simulink model "DC_Virtual_Bus"  (R2025a)
settings: Solver=VariableStepAuto  StartTime=0.0  StopTime=0.8  RelTol=1e-3
libraries: spsIGBTDiodeLib x5, spsSeriesRLCBranchLib x5, spsVoltageMeasurementLib x2, spsDCVoltageSourceLib x1, spsCurrentMeasurementLib x1, simulink x1, sps_lib x1
settings Model: Creator=Mohamed Ibrahim  LastModifiedBy=Mohamed Ibrahim
settings SolverCC: ZeroCrossAlgorithm=Adaptive
settings DebuggingCC: IgnoredZcDiagnostic=none

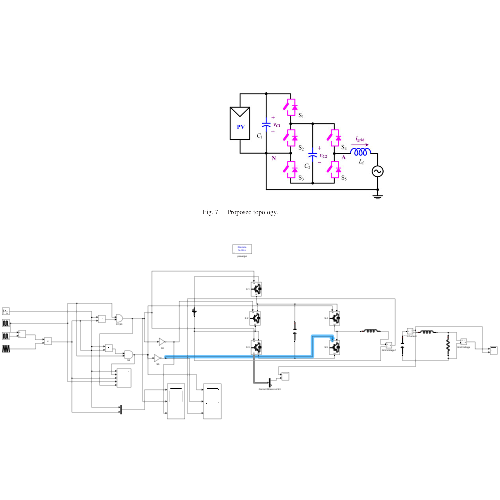
[thumbnail: Simulink's stored preview of the top-level diagram]
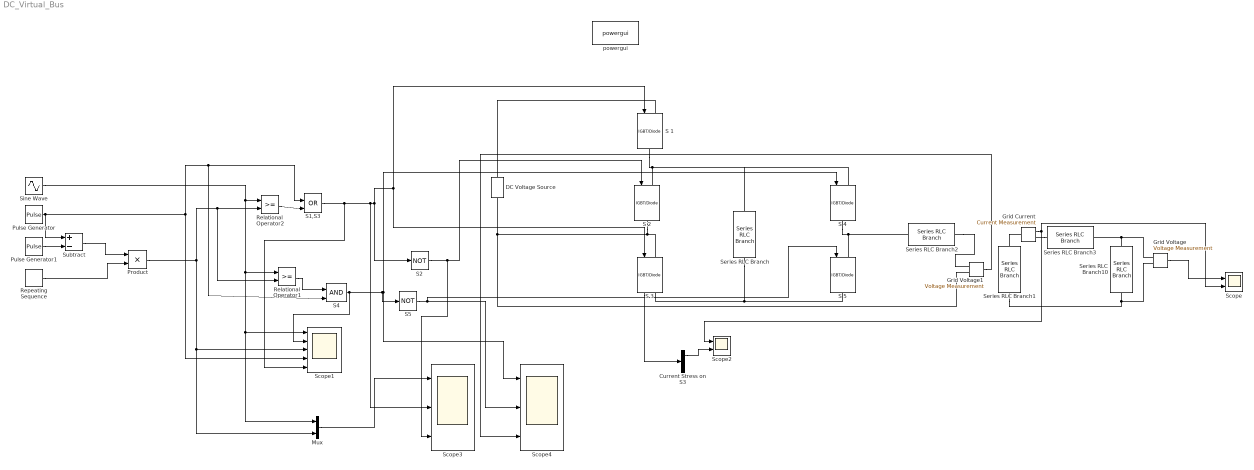
== system DC_Virtual_Bus ==
  Current Stress on S3 : Demux  Outputs=2
  DC Voltage Source : spsDCVoltageSourceLib/DC Voltage Source  Amplitude=400  Measurements=None
  Grid Current : spsCurrentMeasurementLib/Current Measurement  PhasorSimulation=off  OutputType=Complex  PSBequivalent=0
  Grid Voltage : spsVoltageMeasurementLib/Voltage Measurement  PhasorSimulation=off  OutputType=Complex  PSBequivalent=0
  Grid Voltage1 : spsVoltageMeasurementLib/Voltage Measurement  PhasorSimulation=off  OutputType=Complex  PSBequivalent=0
  Mux : Mux  Inputs=2
  Product : Product
  Pulse Generator : DiscretePulseGenerator  PulseType=Time based  Period=0.02  PulseWidth=50
  Pulse Generator1 : DiscretePulseGenerator  PulseType=Time based  Period=0.02  PulseWidth=50  PhaseDelay=0.01
  Relational Operator1 : RelationalOperator  OutDataTypeStr=boolean  RndMeth=Simplest  InputSameDT=off
  Relational Operator2 : RelationalOperator  OutDataTypeStr=boolean  RndMeth=Simplest  InputSameDT=off
  Repeating Sequence : simulink/Sources/Repeating Sequence  rep_seq_t=[0 0.000025 0.00005]  rep_seq_y=[0 1 0]
  S {1..2,4..5} (4 alike) : spsIGBTDiodeLib/IGBT//Diode  Ron=1e-3  Rs=1e5  Cs=inf  Measurements=off
  S 3 : spsIGBTDiodeLib/IGBT//Diode  Ron=1e-3  Rs=1e5  Cs=inf  Measurements=on
  S1,S3 : Logic  Operator=OR  IconShape=distinctive  AllPortsSameDT=off  OutDataTypeStr=boolean
  S2 : Logic  Operator=NOT  IconShape=distinctive  AllPortsSameDT=off  OutDataTypeStr=boolean
  S4 : Logic  IconShape=distinctive  AllPortsSameDT=off  OutDataTypeStr=boolean
  S5 : Logic  Operator=NOT  IconShape=distinctive  AllPortsSameDT=off  OutDataTypeStr=boolean
  Scope : Scope  NumInputPorts=2
      settings: ActiveDisplayYMinimum=-47.58360382260738  ActiveDisplayYMaximum=47.961593181546164
  Scope1 : Scope  NumInputPorts=5
      settings: ActiveDisplayString=4  ActiveDisplayYMinimum=-0.12499999999999997  ActiveDisplayYMaximum=1.125
  Scope2 : Scope  NumInputPorts=2
      settings: ActiveDisplayYMinimum=-47.58360382260738  ActiveDisplayYMaximum=47.961593181546164  DataLoggingVariableName=ScopeData2
  Scope3 : Scope  NumInputPorts=3
      settings: ActiveDisplayYMinimum=-1.25  ActiveDisplayYMaximum=1.25  DataLoggingVariableName=ScopeData3
  Scope4 : Scope  NumInputPorts=3
      settings: ActiveDisplayYMinimum=-0.12499999999999997  ActiveDisplayYMaximum=1.125  DataLoggingVariableName=ScopeData4
  Series RLC Branch : spsSeriesRLCBranchLib/Series RLC Branch  LConnTagsString=__new0  RConnTagsString=__new0  BranchType=C  Resistance=1  Inductance=1e-3  SetiL0=off  InitialCurrent=0  Capacitance=940e-6  Setx0=off  InitialVoltage=0  Measurements=None
  Series RLC Branch1 : spsSeriesRLCBranchLib/Series RLC Branch  LConnTagsString=__new0  RConnTagsString=__new0  BranchType=C  Resistance=1  Inductance=8e-3  SetiL0=off  InitialCurrent=0  Capacitance=0.34e-6  Setx0=off  InitialVoltage=0  Measurements=None
  Series RLC Branch10 : spsSeriesRLCBranchLib/Series RLC Branch  LConnTagsString=__new0  RConnTagsString=__new0  BranchType=R  Resistance=10  Inductance=0.8e-3  SetiL0=off  InitialCurrent=0  Capacitance=1e-6  Setx0=off  InitialVoltage=0  Measurements=None
  Series RLC Branch2 : spsSeriesRLCBranchLib/Series RLC Branch  LConnTagsString=__new0  RConnTagsString=__new0  BranchType=L  Resistance=1  Inductance=8e-3  SetiL0=off  InitialCurrent=0  Capacitance=1e-6  Setx0=off  InitialVoltage=0  Measurements=None
  Series RLC Branch3 : spsSeriesRLCBranchLib/Series RLC Branch  LConnTagsString=__new0  RConnTagsString=__new0  BranchType=L  Resistance=1  Inductance=0.8e-3  SetiL0=off  InitialCurrent=0  Capacitance=1e-6  Setx0=off  InitialVoltage=0  Measurements=None
  Sine Wave : Sin  Frequency=100*pi  SampleTime=0
  Subtract : Sum  Inputs=+-
  powergui : sps_lib/powergui  Priority=1  SimulationMode=Discrete  SampleTime=1e-6  frequency=60  Iterations=50  frequencyindice=0  Pbase=100e6  ErrMax=1e-4  UnitsV=kV  UnitsW=MW  buscounter=0  FunctionMessages=off  echomessages=off  EnableUseOfTLC=off  CurrentSourceSwitches=off  DisableSnubberDevices=off  DisableRonSwitches=off  DisableVfSwitches=off  DisplayEquations=off  AutomaticDiscreteSolvers=off  SolverType=Tustin/Backward Euler (TBE)  Interpol=off  ExternalGateDelay=off  methode=off  Ts=100  x0status=blocks  SPID=on  SwTol=0  HookPort=off  NonlinearTolerance=1e-4  nMaxIteration=100  ContinueOnMaxIteration=off  RestoreLinks=warning  ResistiveCurrentMeasurement=off  Frange=[0:2:500]  Ylog=off  Xlog=on  ShowGrid=off  save=off  variable=ZData  structure=0  ZoomFFT=off  StartTime=0.0  cycles=1  DisplayStyle=1  fundamental=60  FreqAxis=off  MaxFrequency=1000  frequencyindicesteady=1  RmsSteady=1  display=off
  wires:
  Grid Voltage/1 -> Scope/1
  S1,S3/1 -> Scope3/2, S2/1, S 1/1, S 3/1, Scope1/5
  S2/1 -> Scope3/3, S 2/1
  S4/1 -> Scope1/2, Scope4/1, S 4/1, S5/1
  S5/1 -> Scope4/2, S 5/1
  Sine Wave/1 -> Mux/1, Scope1/1, Relational Operator1/1, Relational Operator2/1
  Pulse Generator/1 -> Subtract/1, S4/2, S1,S3/1, Scope1/4
  Relational Operator2/1 -> S1,S3/2
  Relational Operator1/1 -> S4/1
  Product/1 -> Mux/2, Scope1/3, Relational Operator1/2, Relational Operator2/2
  Grid Current/1 -> Scope2/1, Scope/2
  S 3/1 -> Current Stress on S3/1
  Pulse Generator1/1 -> Subtract/2
  Subtract/1 -> Product/1
  Repeating Sequence/1 -> Product/2
  Current Stress on S3/1 -> Scope2/2
  Mux/1 -> Scope3/1
  Grid Voltage1/1 -> Scope4/3
  connections:
  S 1/LConn1 -- DC Voltage Source/RConn1
  S 1/RConn1 -- S 4/LConn1 -- Series RLC Branch/LConn1 -- S 2/LConn1
  Series RLC Branch/RConn1 -- S 5/RConn1 -- S 3/RConn1
  S 4/RConn1 -- Series RLC Branch2/LConn1 -- S 5/LConn1
  Series RLC Branch2/RConn1 -- Grid Voltage1/LConn1
  Grid Voltage/LConn1 -- Series RLC Branch3/RConn1 -- Series RLC Branch10/LConn1
  Grid Current/RConn1 -- Series RLC Branch3/LConn1
  Series RLC Branch1/RConn1 -- Grid Voltage/LConn2 -- Series RLC Branch10/RConn1
  Grid Current/LConn1 -- Series RLC Branch1/LConn1
  S 2/RConn1 -- Grid Voltage1/LConn2 -- DC Voltage Source/LConn1 -- S 3/LConn1
